simulink model "Single_Phase_CHB_Rectifier_Digital_PR"  (R2023b)
settings: Solver=VariableStepAuto  StartTime=0.0  StopTime=0.5  RelTol=1e-3
libraries: spsSeriesRLCBranchLib x6, spsVoltageMeasurementLib x4, spsUniversalBridgeLib x2, spsACVoltageSourceLib x1, spsMeanLib x1, slpidlib x1, powerlib_extras x1, spsRMSLib x1, simulink x1, spsTHDLib x1, spspowerguiLib x1, spsCurrentMeasurementLib x1
settings Model: SimulationMode=accelerator  Creator=abc6820292  LastModifiedBy=Qu
settings DebuggingCC: UnconnectedInputMsg=warning  UnconnectedOutputMsg=warning  UnconnectedLineMsg=warning
settings ModelReferenceCC: EnableRefExpFcnMdlSchedulingChecks=on
settings RTWCC: DLArmComputeVersion=19.05

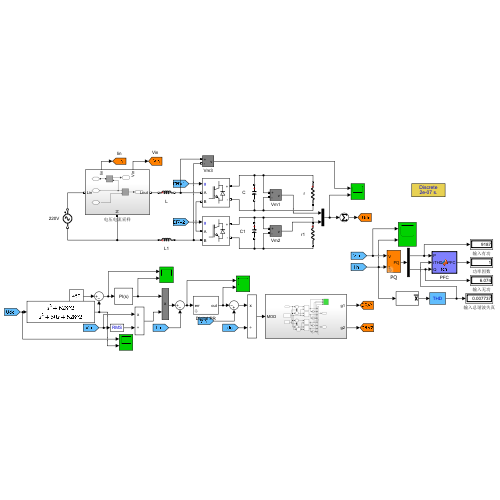
[thumbnail: Simulink's stored preview of the top-level diagram]
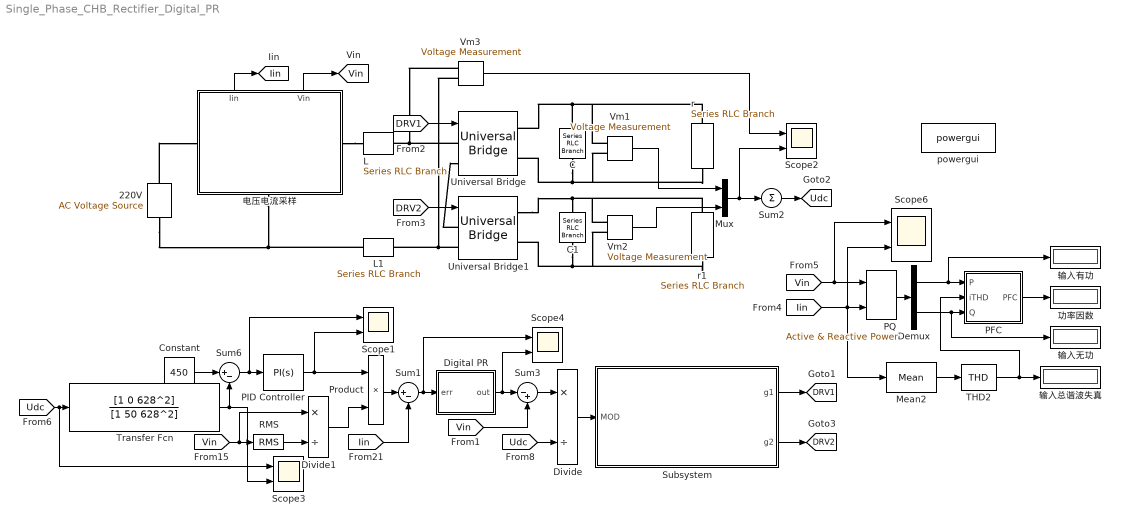
== system Single_Phase_CHB_Rectifier_Digital_PR ==
  220V : spsACVoltageSourceLib/AC Voltage Source  Amplitude=311  Phase=0  Frequency=50  SampleTime=0  Measurements=None  BusType=swing  Pref=10e3  Qref=0  Qmin=-inf  Qmax=+inf
  C : spsSeriesRLCBranchLib/Series RLC Branch  LConnTagsString=__new0  RConnTagsString=__new0  BranchType=C  Resistance=0  Inductance=0  SetiL0=off  InitialCurrent=0  Capacitance=1e-3  Setx0=on  InitialVoltage=155  Measurements=None
  C1 : spsSeriesRLCBranchLib/Series RLC Branch  LConnTagsString=__new0  RConnTagsString=__new0  BranchType=C  Resistance=0  Inductance=0  SetiL0=off  InitialCurrent=0  Capacitance=1e-3  Setx0=on  InitialVoltage=155  Measurements=None
  Constant : Constant  Value=450
  Demux : Demux  Outputs=2
  Digital PR : Subsystem  mask{Kp=6, Kr=100, Wc=5, Ts=1/40000, Upper=400, Lower=-400}
      mask DialogControl ParameterGroupVar Prompt: 参数
  Divide : Product  Inputs=*/
  Divide1 : Product  Inputs=*/
  L : spsSeriesRLCBranchLib/Series RLC Branch  LConnTagsString=__new0  RConnTagsString=__new0  BranchType=L  Resistance=0.1  Inductance=2e-4  SetiL0=off  InitialCurrent=0  Capacitance=inf  Setx0=off  InitialVoltage=0  Measurements=None
  L1 : spsSeriesRLCBranchLib/Series RLC Branch  LConnTagsString=__new0  RConnTagsString=__new0  BranchType=L  Resistance=0.1  Inductance=2e-4  SetiL0=off  InitialCurrent=0  Capacitance=inf  Setx0=off  InitialVoltage=0  Measurements=None
  Mean2 : spsMeanLib/Mean  Freq=5000  Vinit=0  Ts=0
  Mux : Mux  Inputs=2
  PFC : MATLAB Function  TreatAsAtomicUnit=on
  PID Controller : slpidlib/PID Controller  Controller=PI  Form=Parallel  TimeDomain=Continuous-time  UseExternalTs=off  SampleTime=-1  IntegratorMethod=Forward Euler  FilterMethod=Forward Euler  ControllerParametersSource=internal  P=0.15  I=20  UseKiTs=off  D=0.005  N=100  UseFilter=on  TunerSelectOption=Transfer Function Based (PID Tuner App)  InitialConditionSource=internal  InitialConditionForIntegrator=0  InitialConditionForFilter=0  DifferentiatorICPrevScaledInput=0  ExternalReset=none  TrackingMode=off  Kt=1  LimitOutput=off  SatLimitsSource=internal  UpperSaturationLimit=400  LowerSaturationLimit=0  LinearizeAsGain=on  AntiWindupMode=clamping  Kb=1  LimitIntegrator=off  UpperIntegratorSaturationLimit=inf  LowerIntegratorSaturationLimit=-inf  POutMin=[]  POutMax=[]  IOutMin=[]  IOutMax=[]  DOutMin=[]  DOutMax=[]  NOutMin=[]  NOutMax=[]  SumOutMin=[]  SumOutMax=[]  SaturationOutMin=[]  SaturationOutMax=[]  PParamMin=[]  PParamMax=[]  IParamMin=[]  IParamMax=[]  DParamMin=[]  DParamMax=[]  NParamMin=[]  NParamMax=[]  KbParamMin=[]  KbParamMax=[]  KtParamMin=[]  KtParamMax=[]  KbOutMin=[]  KbOutMax=[]  KtOutMin=[]  KtOutMax=[]  IntegratorOutMin=[]  IntegratorOutMax=[]  FilterOutMin=[]  FilterOutMax=[]  SumI1OutMin=[]  SumI1OutMax=[]  SumI2OutMin=[]  SumI2OutMax=[]  SumI3OutMin=[]  SumI3OutMax=[]  SumI4OutMin=[]  SumI4OutMax=[]  SumDOutMin=[]  SumDOutMax=[]  DifferentiatorOutMin=[]  DifferentiatorOutMax=[]  FilterDiffOutCoefMin=[]  FilterDiffOutCoefMax=[]  ReciprocalOutMin=[]  ReciprocalOutMax=[]  SumDenOutMin=[]  SumDenOutMax=[]  SumNumOutMin=[]  SumNumOutMax=[]  DivideOutMin=[]  DivideOutMax=[]  UdiffTsProdOutMin=[]  UdiffTsProdOutMax=[]  NTsProdOutMin=[]  NTsProdOutMax=[]  UintegralTsProdOutMin=[]  UintegralTsProdOutMax=[]  UngainTsProdOutMin=[]  UngainTsProdOutMax=[]  ClampingZeroOutDataTypeStr=Inherit: Inherit via back propagation  ClampingZeroOutMin=[]  ClampingZeroOutMax=[]  FilterDenConstantOutDataTypeStr=Inherit: Inherit via back propagation  FilterDenConstantOutMin=[]  FilterDenConstantOutMax=[]  PCopyOutDataTypeStr=Inherit: Inherit via back propagation  PCopyOutMin=[]  PCopyOutMax=[]  NCopyOutDataTypeStr=Inherit: Inherit via back propagation  NCopyOutMin=[]  NCopyOutMax=[]  IntegratorContinuousStateAttributes=''  IntegratorStateMustResolveToSignalObject=off  IntegratorRTWStateStorageClass=Auto  FilterContinuousStateAttributes=''  FilterStateMustResolveToSignalObject=off  FilterRTWStateStorageClass=Auto  ParallelPVariant=InternalParameters  IdealPVariant=Disabled  IVariant=InternalParameters  DVariant=Disabled  IntegratorVariant=Continuous  SatVariant=Disabled  AWVariant=Passthrough  PCopyVariant=Disabled  TRVariant=Disabled  FdbkBlocksVariant=Forward  IdealPFdbkVariant=Disabled  SatFdbkVariant=Disabled  DerivativeFilterVariant=Disabled  NVariant=Disabled  NCopyVariant=Disabled_SignalSpec  FilterICVariant=Disabled  IntegratorICVariant=InternalICs  ExternalResetVariant=Disabled  TRSumVariant=Passthrough  SumFdbkVariant=Disabled  SumVariant=Sum_PI  TsampFilterVariant=InternalTs  TsampNgainVariant=Passthrough  TsampIntegralVariant=Disabled_SignalSpec  ExternalSaturationOutDataTypeStr=Inherit: Same as second input
  PQ : powerlib_extras/Measurements/Active & Reactive Power  f1=50
  Product : Product  RndMeth=Zero
  RMS : spsRMSLib/RMS  TrueRMS=on  Freq=50  RMSInit=220  Ts=0
  Scope{1..4,6} (5 alike) : Scope  NumInputPorts=2
  Subsystem : Subsystem
  Sum1 : Sum  Inputs=|+-
  Sum2 : Sum  Inputs=+
  Sum3 : Sum  Inputs=|-+
  Sum6 : Sum  Inputs=|+-
  THD2 : spsTHDLib/THD  Freq=50  Ts=0
  Transfer Fcn : TransferFcn  Numerator=[1 0 628^2]  Denominator=[1 50 628^2]
  Universal Bridge : spsUniversalBridgeLib/Universal Bridge  Arms=2  SnubberResistance=1e5  SnubberCapacitance=inf  Device=IGBT / Diodes  Ron=1e-3  Lon=0  ForwardVoltages="[  1  1  ]"  ForwardVoltage=0  GTOparameters=[ 10e-6 , 20e-6 ]  IGBTparameters=[ 1e-6 , 2e-6 ]  Measurements=None  Measurements_2=None  converterType=Rectifier
  Universal Bridge1 : spsUniversalBridgeLib/Universal Bridge  Arms=2  SnubberResistance=1e5  SnubberCapacitance=inf  Device=IGBT / Diodes  Ron=1e-3  Lon=0  ForwardVoltages="[  1  1  ]"  ForwardVoltage=0  GTOparameters=[ 10e-6 , 20e-6 ]  IGBTparameters=[ 1e-6 , 2e-6 ]  Measurements=None  Measurements_2=None  converterType=Rectifier
  Vm1 : spsVoltageMeasurementLib/Voltage Measurement  PhasorSimulation=off  OutputType=Complex  PSBequivalent=0
  Vm2 : spsVoltageMeasurementLib/Voltage Measurement  PhasorSimulation=off  OutputType=Complex  PSBequivalent=0
  Vm3 : spsVoltageMeasurementLib/Voltage Measurement  PhasorSimulation=off  OutputType=Complex  PSBequivalent=0
  powergui : spspowerguiLib/powergui  SimulationMode=Discrete  SampleTime=2e-7  frequency=60  Iterations=50  frequencyindice=0  Pbase=100e6  ErrMax=1e-4  UnitsV=kV  UnitsW=MW  buscounter=0  FunctionMessages=off  echomessages=off  EnableUseOfTLC=off  CurrentSourceSwitches=off  DisableSnubberDevices=off  DisableRonSwitches=off  DisableVfSwitches=off  DisplayEquations=off  AutomaticDiscreteSolvers=off  SolverType=Tustin/Backward Euler (TBE)  Interpol=off  ExternalGateDelay=off  methode=off  Ts=0  x0status=blocks  SPID=off  SwTol=0  HookPort=off  NonlinearTolerance=1e-4  nMaxIteration=100  ContinueOnMaxIteration=off  RestoreLinks=warning  ResistiveCurrentMeasurement=off  Frange=[0:2:500]  Ylog=off  Xlog=on  ShowGrid=off  save=off  variable=ZData  structure=QQQQQ  ZoomFFT=off  StartTime=0.5  cycles=15  DisplayStyle=1  fundamental=50  FreqAxis=off  MaxFrequency=1000  frequencyindicesteady=1  RmsSteady=1  display=off
  r : spsSeriesRLCBranchLib/Series RLC Branch  LConnTagsString=__new0  RConnTagsString=__new0  BranchType=R  Resistance=30  Inductance=12e-4  SetiL0=off  InitialCurrent=0  Capacitance=inf  Setx0=off  InitialVoltage=0  Measurements=None
  r1 : spsSeriesRLCBranchLib/Series RLC Branch  LConnTagsString=__new0  RConnTagsString=__new0  BranchType=R  Resistance=30  Inductance=12e-4  SetiL0=off  InitialCurrent=0  Capacitance=inf  Setx0=off  InitialVoltage=0  Measurements=None
  功率因数 : Display
  电压电流采样 : Subsystem
      settings: PortSchema="{\"entries\":[{\"content\":{\"sides\":[{\"content\":{\"connectorIds\":[\"LConn1\"]},\"type\":\"ConnectorPlacement.EquallySpacedRectSide\",\"uuid\":\"d60dd16a-7a74-435a-96f5-79c0993f3801\"},{\"content\":{\"connectorIds\":[\"RConn1\"],\"side\":\"RIGHT\"},\"type\":\"ConnectorPlacement.EquallySpacedRectSide\",\"uuid\":\"38a0d536-50a5-43bd-9d58-6b0db9c378a0\"},{\"content\":{\"connectorIds\":[\"Out1\",\"Out2\"],\"side\":\"TOP\"},\"type\":\"ConnectorPlacement.EquallySpacedRectSide\",\"uuid\":\"65be575f-dbb8-4f94-beb1-b426df65c1d5\"},{\"content\":{\"connectorIds\":[\"RConn2\"],\"side\":\"BOTTOM\"},\"type\":\"ConnectorPlacement.EquallySpacedRectSide\",\"uuid\":\"a28dffe8-15db-4523-b673-2414d0fbe1e1\"}]},\"type\":\"ConnectorPlacement.EquallySpacedConnector\",\"uuid\":\"1fc3ca7a-50b1-4fd5-a5d3-d39cc1e6f07d\"}],\"packageUris\":[\"http://schema.mathworks.com/mf0/Connector/R2020b\"],\"version\":\"1.0\"}"
  输入总谐波失真 : Display
  输入无功 : Display
  输入有功 : Display
  tag scope: DRV1=global, DRV2=global, Iin=global, Udc=global, Vin=global
  wires:
  电压电流采样/2(Vin) -> [Vin]
  电压电流采样/1(Iin) -> [Iin]
  Sum6/1 -> PID Controller/1, Scope1/1
  PID Controller/1 -> Product/1, Scope1/2
  Vm1/1 -> Mux/1
  Vm2/1 -> Mux/2
  [DRV1] -> Universal Bridge/1
  [DRV2] -> Universal Bridge1/1
  Sum1/1 -> Scope4/1, Digital PR/1(err)
  Product/1 -> Sum1/1
  Constant/1 -> Sum6/1
  [Iin] -> Sum1/2
  Digital PR/1(out) -> Sum3/1, Scope4/2
  [Vin] -> Sum3/2
  Sum3/1 -> Divide/1
  [Udc] -> Divide/2
  Sum2/1 -> [Udc]
  Mux/1 -> Sum2/1, Scope2/2
  [Vin] -> Divide1/1, RMS/1
  RMS/1 -> Divide1/2
  Divide1/1 -> Product/2
  Divide/1 -> Subsystem/1(MOD)
  Subsystem/1(g1) -> [DRV1]
  Subsystem/2(g2) -> [DRV2]
  THD2/1 -> 输入总谐波失真/1, PFC/2(iTHD)
  Demux/2 -> 输入无功/1, PFC/3(Q)
  PFC/1(PFC) -> 功率因数/1
  [Vin] -> PQ/1, Scope6/1
  PQ/1 -> Demux/1
  Mean2/1 -> THD2/1
  [Iin] -> Mean2/1, Scope6/2, PQ/2
  Demux/1 -> 输入有功/1, PFC/1(P)
  Vm3/1 -> Scope2/1
  [Udc] -> Scope3/1, Transfer Fcn/1
  Transfer Fcn/1 -> Scope3/2, Sum6/2
  connections:
  电压电流采样/RConn2 -- 220V/LConn1 -- L1/LConn1
  电压电流采样/RConn1 -- L/LConn1
  Universal Bridge/LConn1 -- Vm3/LConn1 -- L/RConn1
  Universal Bridge1/LConn2 -- Vm3/LConn2 -- L1/RConn1
  220V/RConn1 -- 电压电流采样/LConn1
  Universal Bridge1/LConn1 -- Universal Bridge/LConn2
  C/LConn1 -- r/LConn1 -- Vm1/LConn1 -- Universal Bridge/RConn1
  C/RConn1 -- r/RConn1 -- Vm1/LConn2 -- Universal Bridge/RConn2
  Universal Bridge1/RConn1 -- r1/LConn1 -- Vm2/LConn1 -- C1/LConn1
  C1/RConn1 -- r1/RConn1 -- Vm2/LConn2 -- Universal Bridge1/RConn2

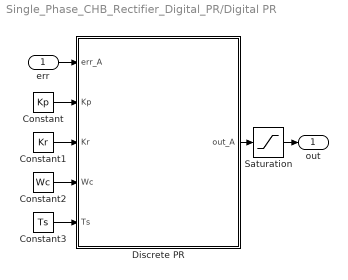
== system Single_Phase_CHB_Rectifier_Digital_PR/Digital PR ==
  err : Inport
  Constant : Constant  Value=Kp
  Constant1 : Constant  Value=Kr
  Constant2 : Constant  Value=Wc
  Constant3 : Constant  Value=Ts
  Discrete PR : MATLAB Function  TreatAsAtomicUnit=on
  Saturation : Saturate  UpperLimit=Upper  LowerLimit=Lower
  out : Outport
  wires:
  Constant1/1 -> Discrete PR/3(Kr)
  Constant3/1 -> Discrete PR/5(Ts)
  Constant/1 -> Discrete PR/2(Kp)
  Constant2/1 -> Discrete PR/4(Wc)
  Discrete PR/1(out_A) -> Saturation/1
  Saturation/1 -> out/1
  err/1 -> Discrete PR/1(err_A)

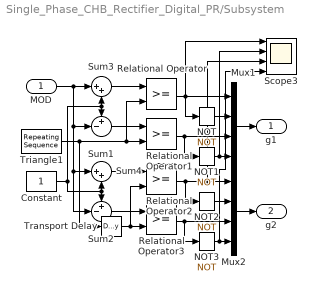
== system Single_Phase_CHB_Rectifier_Digital_PR/Subsystem ==
  MOD : Inport
  Constant : Constant
  Mux1 : Mux
  Mux2 : Mux
  NOT{,1..3} (4 alike) : Logic  Operator=NOT  IconShape=distinctive  AllPortsSameDT=off  OutDataTypeStr=boolean
  Relational Operator{,1..3} (4 alike) : RelationalOperator  OutDataTypeStr=boolean  InputSameDT=off
  Scope3 : Scope  NumInputPorts=4
  Sum1 : Sum  Inputs=+-|
  Sum2 : Sum  Inputs=+-|
  Sum3 : Sum  Inputs=|++
  Sum4 : Sum  Inputs=|++
  Transport Delay : TransportDelay  DelayTime=1/10000/4
  Triangle1 : simulink/Sources/Repeating Sequence  rep_seq_t=[0 1/10000/2 1/10000]  rep_seq_y=[0 2 0]
  g1 : Outport
  g2 : Outport  Port=2
  wires:
  Mux1/1 -> g1/1
  MOD/1 -> Sum2/2, Sum4/1, Sum1/2, Sum3/1
  Relational Operator/1 -> Scope3/1, NOT/1, Mux1/1
  NOT/1 -> Mux1/2
  NOT1/1 -> Scope3/2, Mux1/4
  Relational Operator1/1 -> NOT1/1, Mux1/3
  Sum3/1 -> Relational Operator/1
  Triangle1/1 -> Transport Delay/1, Relational Operator1/2, Relational Operator/2
  Sum1/1 -> Relational Operator1/1
  Sum2/1 -> Relational Operator3/1
  Sum4/1 -> Relational Operator2/1
  Relational Operator3/1 -> Mux2/3, NOT3/1
  NOT3/1 -> Scope3/4, Mux2/4
  NOT2/1 -> Mux2/2
  Relational Operator2/1 -> Mux2/1, Scope3/3, NOT2/1
  Mux2/1 -> g2/1
  Constant/1 -> Sum2/1, Sum4/2, Sum3/2, Sum1/1
  Transport Delay/1 -> Relational Operator2/2, Relational Operator3/2

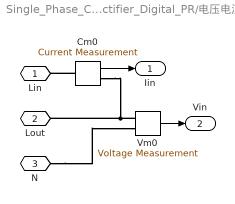
== system Single_Phase_CHB_Rectifier_Digital_PR/电压电流采样 ==
  Cm0 : spsCurrentMeasurementLib/Current Measurement  PhasorSimulation=off  OutputType=Complex  PSBequivalent=0
  Vm0 : spsVoltageMeasurementLib/Voltage Measurement  PhasorSimulation=off  OutputType=Complex  PSBequivalent=0
  Lin : PMIOPort  Side=Left
  Lout : PMIOPort  Port=2  Side=Right
  N : PMIOPort  Port=3  Side=Right
  Iin : Outport
  Vin : Outport  Port=2
  wires:
  Cm0/1 -> Iin/1
  Vm0/1 -> Vin/1
  connections:
  Cm0/RConn1 -- Vm0/LConn1 -- Lout/RConn1
  Cm0/LConn1 -- Lin/RConn1
  N/RConn1 -- Vm0/LConn2

== matlab function Single_Phase_CHB_Rectifier_Digital_PR/PFC ==
  data: P input; iTHD input; PFC output; Q input
function PFC = fcn(P,iTHD,Q)
% This block supports an embeddable subset of the MATLAB language.
% See the help menu for details. 
PFC=(P/sqrt(P*P+Q*Q))/sqrt(1+iTHD*iTHD);

== matlab function Single_Phase_CHB_Rectifier_Digital_PR/Digital PR/Discrete PR ==
  settings: updateMethod=DISCRETE  sampleTime=Ts
  data: err_A input; out_A output; Kp input; Kr input; Wc input; Ts input
function out_A  = fcn(err_A, Kp, Kr, Wc, Ts)

W0 = 50*2*pi;


persistent err_A1;
persistent err_A2;
persistent out_A1;
persistent out_A2;


%%对三相静态变量初始化
if isempty(err_A1)
    err_A1 = 0;
end
if isempty(err_A2)
    err_A2 = 0;
end
if isempty(out_A1)
    out_A1 = 0;
end
if isempty(out_A2)
    out_A2 = 0;
end


%%Discrete
t1 = Wc * Ts;
t2 = W0^2 * Ts^2;
t3 = t2 + 4*t1 + 4;

b0 = (Kp*t2 + 4*(Kp+Kr)*t1 + 4*Kp) / t3;
b1 = (2*Kp*t2 - 8*Kp) / t3;
b2 = (Kp*t2 + 4*Kp - 4*(Kp+Kr)*t1) / t3;
a1 = (2*t2 - 8) / t3;
a2 = (t2 - 4*t1 + 4) / t3;
%%限制输出
if b0>3000
    b0=0;
end
if b0<-3000
    b0=0;
end

%%计算输出量
out_A = b0*err_A + b1*err_A1 + b2*err_A2 - a1*out_A1 - a2*out_A2;
out_A2 = out_A1;
out_A1 = out_A;
err_A2 = err_A1;
err_A1 = err_A;
